simulink model "DC_Microgrid_Solar_Battery_Simulink"  (R2025b)
settings: Solver=ode1  StartTime=0.0  StopTime=25.0  FixedStep=0.01  RelTol=1e-3
InitFcn:
  | startup;
StopFcn:
  | run_solar_battery_microgrid_benchmark;
undefined symbols (not defined in the file): DiscIntNeverNeededParam
libraries: slpidlib x1, simulink x1
settings Model: Creator=Santhosh  LastModifiedBy=Santhosh

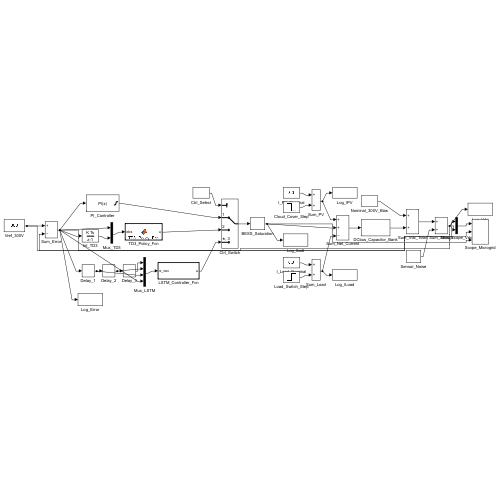
[thumbnail: Simulink's stored preview of the top-level diagram]
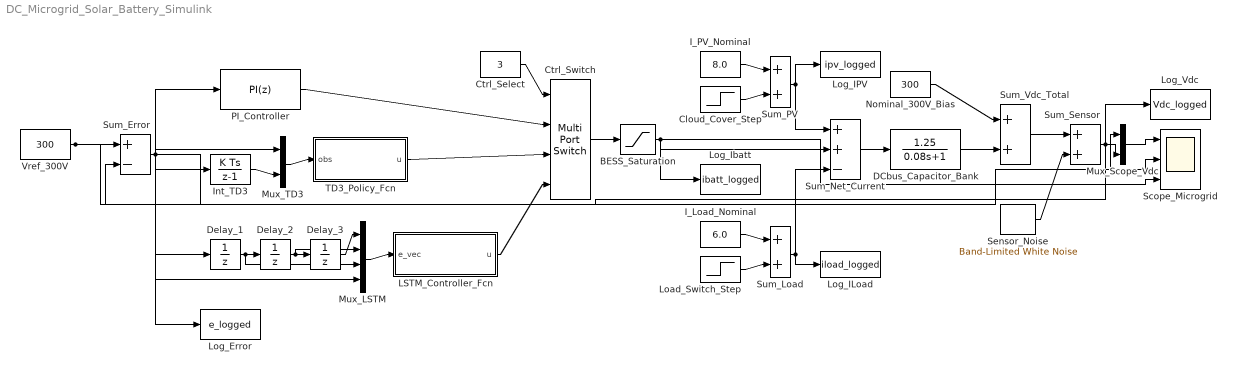
== system DC_Microgrid_Solar_Battery_Simulink ==
  BESS_Saturation : Saturate  UpperLimit=10.0503  LowerLimit=-9.33386
  Cloud_Cover_Step : Step  Time=8.0  After=-4.0  SampleTime=0.01
  Ctrl_Select : Constant  Value=3
  Ctrl_Switch : MultiPortSwitch  SaturateOnIntegerOverflow=off  InputSameDT=off
  DCbus_Capacitor_Bank : TransferFcn  Numerator=[1.25]  Denominator=[0.08 1]
  Delay_1 : UnitDelay  SampleTime=0.01  HasFrameUpgradeWarning=on
  Delay_2 : UnitDelay  SampleTime=0.01  HasFrameUpgradeWarning=on
  Delay_3 : UnitDelay  SampleTime=0.01  HasFrameUpgradeWarning=on
  I_Load_Nominal : Constant  Value=6.0
  I_PV_Nominal : Constant  Value=8.0
  Int_TD3 : DiscreteIntegrator  SampleTime=0.01  ICPrevOutput=DiscIntNeverNeededParam  ICPrevScaledInput=DiscIntNeverNeededParam
  LSTM_Controller_Fcn : MATLAB Function  TreatAsAtomicUnit=on
  Load_Switch_Step : Step  Time=16.0  After=6.5  SampleTime=0.01
  Log_Error : ToWorkspace  VariableName=e_logged  SampleTime=-1
  Log_ILoad : ToWorkspace  VariableName=iload_logged  SampleTime=-1
  Log_IPV : ToWorkspace  VariableName=ipv_logged  SampleTime=-1
  Log_Ibatt : ToWorkspace  VariableName=ibatt_logged  SampleTime=-1
  Log_Vdc : ToWorkspace  VariableName=Vdc_logged  SampleTime=-1
  Mux_LSTM : Mux
  Mux_Scope_Vdc : Mux  Inputs=2
  Mux_TD3 : Mux  Inputs=2
  Nominal_300V_Bias : Constant  Value=300
  PI_Controller : slpidlib/PID Controller  Controller=PI  Form=Parallel  TimeDomain=Discrete-time  UseExternalTs=off  SampleTime=0.01  IntegratorMethod=Forward Euler  FilterMethod=Forward Euler  ControllerParametersSource=internal  P=0.85  I=1.20  UseKiTs=off  D=0  UseExternalDerivativeSource=off  N=100  UseFilter=on  TunerSelectOption=Transfer Function Based (PID Tuner App)  InitialConditionSource=internal  InitialConditionForIntegrator=0  InitialConditionForFilter=0  DifferentiatorICPrevScaledInput=0  ExternalReset=none  TrackingMode=off  Kt=1  LimitOutput=on  SatLimitsSource=internal  UpperSaturationLimit=10.0503  LowerSaturationLimit=-9.33386  LinearizeAsGain=on  AntiWindupMode=none  Kb=1  LimitIntegrator=off  UpperIntegratorSaturationLimit=inf  LowerIntegratorSaturationLimit=-inf  POutMin=[]  POutMax=[]  IOutMin=[]  IOutMax=[]  DOutMin=[]  DOutMax=[]  NOutMin=[]  NOutMax=[]  SumOutMin=[]  SumOutMax=[]  SaturationOutMin=[]  SaturationOutMax=[]  PParamMin=[]  PParamMax=[]  IParamMin=[]  IParamMax=[]  DParamMin=[]  DParamMax=[]  NParamMin=[]  NParamMax=[]  KbParamMin=[]  KbParamMax=[]  KtParamMin=[]  KtParamMax=[]  KbOutMin=[]  KbOutMax=[]  KtOutMin=[]  KtOutMax=[]  IntegratorOutMin=[]  IntegratorOutMax=[]  FilterOutMin=[]  FilterOutMax=[]  SumI1OutMin=[]  SumI1OutMax=[]  SumI2OutMin=[]  SumI2OutMax=[]  SumI3OutMin=[]  SumI3OutMax=[]  SumI4OutMin=[]  SumI4OutMax=[]  SumDOutMin=[]  SumDOutMax=[]  DifferentiatorOutMin=[]  DifferentiatorOutMax=[]  FilterDiffOutCoefMin=[]  FilterDiffOutCoefMax=[]  ReciprocalOutMin=[]  ReciprocalOutMax=[]  SumDenOutMin=[]  SumDenOutMax=[]  SumNumOutMin=[]  SumNumOutMax=[]  DivideOutMin=[]  DivideOutMax=[]  UdiffTsProdOutMin=[]  UdiffTsProdOutMax=[]  NTsProdOutMin=[]  NTsProdOutMax=[]  UintegralTsProdOutMin=[]  UintegralTsProdOutMax=[]  UngainTsProdOutMin=[]  UngainTsProdOutMax=[]  ClampingZeroOutDataTypeStr=Inherit: Inherit via back propagation  ClampingZeroOutMin=[]  ClampingZeroOutMax=[]  FilterDenConstantOutDataTypeStr=Inherit: Inherit via back propagation  FilterDenConstantOutMin=[]  FilterDenConstantOutMax=[]  PCopyOutDataTypeStr=Inherit: Inherit via back propagation  PCopyOutMin=[]  PCopyOutMax=[]  NCopyOutDataTypeStr=Inherit: Inherit via back propagation  NCopyOutMin=[]  NCopyOutMax=[]  IntegratorContinuousStateAttributes=''  IntegratorStateMustResolveToSignalObject=off  IntegratorRTWStateStorageClass=Auto  FilterContinuousStateAttributes=''  FilterStateMustResolveToSignalObject=off  FilterRTWStateStorageClass=Auto  ParallelPVariant=InternalParameters  IdealPVariant=Disabled  IVariant=InternalParameters  DVariant=Disabled  IntegratorVariant=Discrete  SatVariant=Enabled  AWVariant=Passthrough  PCopyVariant=Disabled  TRVariant=Disabled  FdbkBlocksVariant=Forward  IdealPFdbkVariant=Disabled  SatFdbkVariant=Disabled  DerivativeFilterVariant=Disabled  NVariant=Disabled  NCopyVariant=Disabled_SignalSpec  FilterICVariant=Disabled  IntegratorICVariant=InternalICs  ExternalResetVariant=Disabled  TRSumVariant=Passthrough  SumFdbkVariant=Disabled  SumVariant=Sum_PI  TsampFilterVariant=InternalTs  TsampNgainVariant=Passthrough  TsampIntegralVariant=Disabled_SignalSpec  ExternalSaturationOutDataTypeStr=Inherit: Same as second input  DerivativeSourceVariant=Disabled  PreIntVariant=InternalPreInt
  Scope_Microgrid : Scope  NumInputPorts=3
  Sensor_Noise : simulink/Sources/Band-Limited White Noise  Cov=0.005  Ts=0.01  seed=[23341]
  Sum_Error : Sum  Inputs=+-
  Sum_Load : Sum
  Sum_Net_Current : Sum  Inputs=++-
  Sum_PV : Sum
  Sum_Sensor : Sum
  Sum_Vdc_Total : Sum
  TD3_Policy_Fcn : MATLAB Function  TreatAsAtomicUnit=on
  Vref_300V : Constant  Value=300
  wires:
  Vref_300V/1 -> Sum_Error/1, Mux_Scope_Vdc/1
  Sum_Sensor/1 -> Sum_Error/2, Log_Vdc/1, Mux_Scope_Vdc/2
  Mux_Scope_Vdc/1 -> Scope_Microgrid/1
  Sum_Error/1 -> Scope_Microgrid/2, Log_Error/1, PI_Controller/1, Mux_TD3/1, Int_TD3/1, Delay_1/1, Mux_LSTM/4
  BESS_Saturation/1 -> Scope_Microgrid/3, Log_Ibatt/1, Sum_Net_Current/2
  Int_TD3/1 -> Mux_TD3/2
  Mux_TD3/1 -> TD3_Policy_Fcn/1(obs)
  Delay_1/1 -> Delay_2/1, Mux_LSTM/3
  Delay_2/1 -> Delay_3/1, Mux_LSTM/2
  Delay_3/1 -> Mux_LSTM/1
  Mux_LSTM/1 -> LSTM_Controller_Fcn/1(e_vec)
  Ctrl_Select/1 -> Ctrl_Switch/1
  PI_Controller/1 -> Ctrl_Switch/2
  TD3_Policy_Fcn/1(u) -> Ctrl_Switch/3
  LSTM_Controller_Fcn/1(u) -> Ctrl_Switch/4
  Ctrl_Switch/1 -> BESS_Saturation/1
  I_PV_Nominal/1 -> Sum_PV/1
  Cloud_Cover_Step/1 -> Sum_PV/2
  Sum_PV/1 -> Log_IPV/1, Sum_Net_Current/1
  I_Load_Nominal/1 -> Sum_Load/1
  Load_Switch_Step/1 -> Sum_Load/2
  Sum_Load/1 -> Log_ILoad/1, Sum_Net_Current/3
  Sum_Net_Current/1 -> DCbus_Capacitor_Bank/1
  Nominal_300V_Bias/1 -> Sum_Vdc_Total/1
  DCbus_Capacitor_Bank/1 -> Sum_Vdc_Total/2
  Sum_Vdc_Total/1 -> Sum_Sensor/1
  Sensor_Noise/1 -> Sum_Sensor/2

== matlab function DC_Microgrid_Solar_Battery_Simulink/TD3_Policy_Fcn ==
  data: obs input; u output
function u = TD3_Policy_Fcn(obs)
% TD3 Calibrated Actor Policy for BESS Converter
Kp_rl = 1.45;
Ki_rl = 1.85;
e = obs(1);
int_e = obs(2);
u_raw = Kp_rl * e + Ki_rl * int_e;
u = max(min(u_raw, 10.0503), -9.33386);

== matlab function DC_Microgrid_Solar_Battery_Simulink/LSTM_Controller_Fcn ==
  data: e_vec input; u output
function u = LSTM_Controller_Fcn(e_vec)
% Trained 4-Step Memory LSTM Controller Evaluation
coder.extrinsic('evaluate_lstm_controller');
u = 0.0;
u = evaluate_lstm_controller(e_vec);
